simulink model "bb_core"  (R2025b)
settings: Solver=FixedStepDiscrete  StartTime=0.0  StopTime=0.035000000000000003  FixedStep=1/24e6  RelTol=1e-3
model workspace (MAT data in the model file):
  P_ABS_MAX_US = 2600
  P_ABS_MIN_US = 500
  P_CLK_PER_US = 24
  P_CMD = [165 11 0 10 164 165 141 0 0 40 165 0 3 231 64 165 143 0 0 42]
  P_CMD_T0 = 0.0005
  P_DEF_CENTER = 1750
  P_DEF_DSHIFT = 2
  P_DEF_ILIM = 200
  P_DEF_KD = 12800
  P_DEF_KI = 2
  P_DEF_KP = 768
  P_DEF_MANUAL = 1750
  P_DEF_MODE = 13
  P_DEF_SETPOINT = 330
  P_DEF_SMAX = 2500
  P_DEF_SMIN = 1000
  P_DEF_TRIG_MS = 40
  P_DT = 4.16666666667e-08
  P_ECHO_MAX_US = 30000
  P_INIT_US = 1750
  P_MAX_MM = 1000
  P_MIN_MM = 20
  P_MM_PER_US_Q16 = 11239
  P_PERIOD_US = 20000
  P_RISE_TMO_US = 10000
  P_TRIG_US = 12
  P_UART_DIV = 208
  P_VERSION = 47873
settings Model: Creator=Thanotos  LastModifiedBy=Thanotos
settings DebuggingCC: AlgebraicLoopMsg=error  SingleTaskRateTransMsg=error

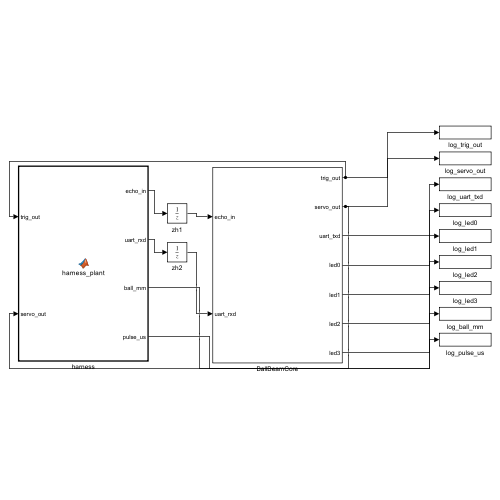
[thumbnail: Simulink's stored preview of the top-level diagram]
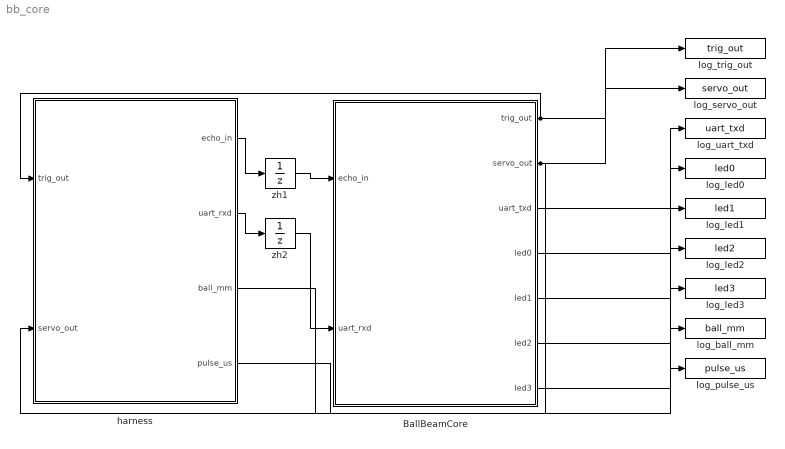
== system bb_core ==
  BallBeamCore : Subsystem
  harness : MATLAB Function  TreatAsAtomicUnit=on
  log_ball_mm : ToWorkspace  VariableName=ball_mm  SampleTime=-1
      settings: Decimation=2400
  log_led0 : ToWorkspace  VariableName=led0  SampleTime=-1
  log_led1 : ToWorkspace  VariableName=led1  SampleTime=-1
  log_led2 : ToWorkspace  VariableName=led2  SampleTime=-1
  log_led3 : ToWorkspace  VariableName=led3  SampleTime=-1
  log_pulse_us : ToWorkspace  VariableName=pulse_us  SampleTime=-1
      settings: Decimation=2400
  log_servo_out : ToWorkspace  VariableName=servo_out  SampleTime=-1
  log_trig_out : ToWorkspace  VariableName=trig_out  SampleTime=-1
  log_uart_txd : ToWorkspace  VariableName=uart_txd  SampleTime=-1
  zh1 : UnitDelay  SampleTime=-1  HasFrameUpgradeWarning=on
  zh2 : UnitDelay  InitialCondition=1  SampleTime=-1  HasFrameUpgradeWarning=on
  wires:
  harness/1(echo_in) -> zh1/1
  zh1/1 -> BallBeamCore/1(echo_in)
  harness/2(uart_rxd) -> zh2/1
  zh2/1 -> BallBeamCore/2(uart_rxd)
  BallBeamCore/1(trig_out) -> harness/1(trig_out), log_trig_out/1
  BallBeamCore/2(servo_out) -> harness/2(servo_out), log_servo_out/1
  BallBeamCore/3(uart_txd) -> log_uart_txd/1
  BallBeamCore/4(led0) -> log_led0/1
  BallBeamCore/5(led1) -> log_led1/1
  BallBeamCore/6(led2) -> log_led2/1
  BallBeamCore/7(led3) -> log_led3/1
  harness/3(ball_mm) -> log_ball_mm/1
  harness/4(pulse_us) -> log_pulse_us/1

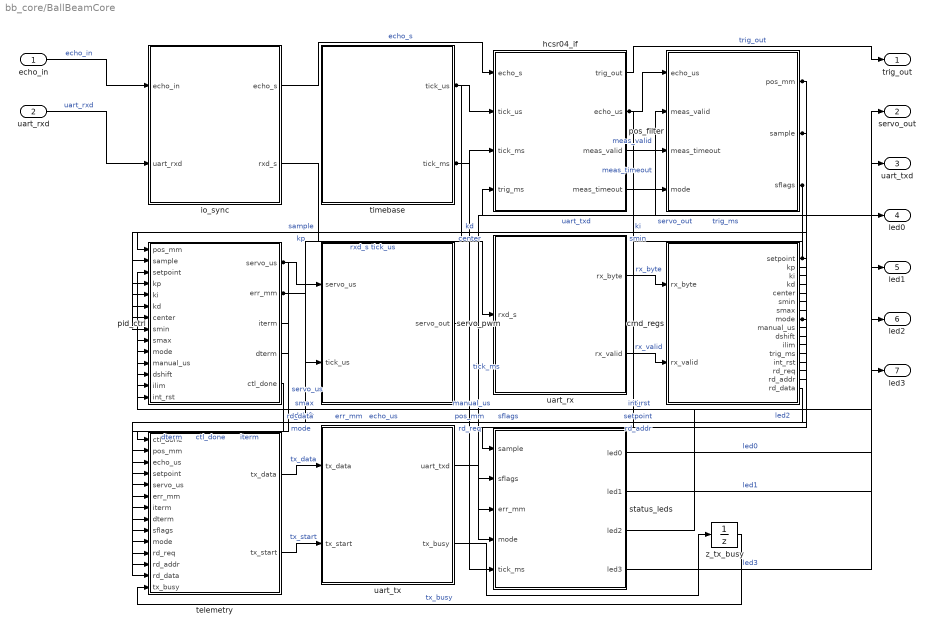
== system bb_core/BallBeamCore ==
  echo_in : Inport  OutDataTypeStr=boolean
  uart_rxd : Inport  Port=2  OutDataTypeStr=boolean
  cmd_regs : MATLAB Function  TreatAsAtomicUnit=on
  hcsr04_if : MATLAB Function  TreatAsAtomicUnit=on
  io_sync : MATLAB Function  TreatAsAtomicUnit=on
  pid_ctrl : MATLAB Function  TreatAsAtomicUnit=on
  pos_filter : MATLAB Function  TreatAsAtomicUnit=on
  servo_pwm : MATLAB Function  TreatAsAtomicUnit=on
  status_leds : MATLAB Function  TreatAsAtomicUnit=on
  telemetry : MATLAB Function  TreatAsAtomicUnit=on
  timebase : MATLAB Function  TreatAsAtomicUnit=on
  uart_rx : MATLAB Function  TreatAsAtomicUnit=on
  uart_tx : MATLAB Function  TreatAsAtomicUnit=on
  z_tx_busy : UnitDelay  SampleTime=-1  HasFrameUpgradeWarning=on
  trig_out : Outport
  servo_out : Outport  Port=2
  uart_txd : Outport  Port=3
  led0 : Outport  Port=4
  led1 : Outport  Port=5
  led2 : Outport  Port=6
  led3 : Outport  Port=7
  wires:
  echo_in/1 -> io_sync/1(echo_in)  "echo_in"
  uart_rxd/1 -> io_sync/2(uart_rxd)  "uart_rxd"
  io_sync/1(echo_s) -> hcsr04_if/1(echo_s)  "echo_s"
  timebase/1(tick_us) -> hcsr04_if/2(tick_us), servo_pwm/2(tick_us)  "tick_us"
  timebase/2(tick_ms) -> hcsr04_if/3(tick_ms), status_leds/5(tick_ms)  "tick_ms"
  cmd_regs/12(trig_ms) -> hcsr04_if/4(trig_ms)  "trig_ms"
  hcsr04_if/2(echo_us) -> pos_filter/1(echo_us), telemetry/3(echo_us)  "echo_us"
  hcsr04_if/3(meas_valid) -> pos_filter/2(meas_valid)  "meas_valid"
  hcsr04_if/4(meas_timeout) -> pos_filter/3(meas_timeout)  "meas_timeout"
  cmd_regs/8(mode) -> pos_filter/4(mode), pid_ctrl/10(mode), telemetry/10(mode), status_leds/4(mode)  "mode"
  pos_filter/1(pos_mm) -> pid_ctrl/1(pos_mm), telemetry/2(pos_mm)  "pos_mm"
  pos_filter/2(sample) -> pid_ctrl/2(sample), status_leds/1(sample)  "sample"
  cmd_regs/1(setpoint) -> pid_ctrl/3(setpoint), telemetry/4(setpoint)  "setpoint"
  cmd_regs/2(kp) -> pid_ctrl/4(kp)  "kp"
  cmd_regs/3(ki) -> pid_ctrl/5(ki)  "ki"
  cmd_regs/4(kd) -> pid_ctrl/6(kd)  "kd"
  cmd_regs/5(center) -> pid_ctrl/7(center)  "center"
  cmd_regs/6(smin) -> pid_ctrl/8(smin)  "smin"
  cmd_regs/7(smax) -> pid_ctrl/9(smax)  "smax"
  cmd_regs/9(manual_us) -> pid_ctrl/11(manual_us)  "manual_us"
  cmd_regs/10(dshift) -> pid_ctrl/12(dshift)  "dshift"
  cmd_regs/11(ilim) -> pid_ctrl/13(ilim)  "ilim"
  cmd_regs/13(int_rst) -> pid_ctrl/14(int_rst)  "int_rst"
  pid_ctrl/1(servo_us) -> servo_pwm/1(servo_us), telemetry/5(servo_us)  "servo_us"
  io_sync/2(rxd_s) -> uart_rx/1(rxd_s)  "rxd_s"
  uart_rx/1(rx_byte) -> cmd_regs/1(rx_byte)  "rx_byte"
  uart_rx/2(rx_valid) -> cmd_regs/2(rx_valid)  "rx_valid"
  pid_ctrl/5(ctl_done) -> telemetry/1(ctl_done)  "ctl_done"
  pid_ctrl/2(err_mm) -> telemetry/6(err_mm), status_leds/3(err_mm)  "err_mm"
  pid_ctrl/3(iterm) -> telemetry/7(iterm)  "iterm"
  pid_ctrl/4(dterm) -> telemetry/8(dterm)  "dterm"
  pos_filter/3(sflags) -> telemetry/9(sflags), status_leds/2(sflags)  "sflags"
  cmd_regs/14(rd_req) -> telemetry/11(rd_req)  "rd_req"
  cmd_regs/15(rd_addr) -> telemetry/12(rd_addr)  "rd_addr"
  cmd_regs/16(rd_data) -> telemetry/13(rd_data)  "rd_data"
  uart_tx/2(tx_busy) -> z_tx_busy/1
  z_tx_busy/1 -> telemetry/14(tx_busy)  "tx_busy"
  telemetry/1(tx_data) -> uart_tx/1(tx_data)  "tx_data"
  telemetry/2(tx_start) -> uart_tx/2(tx_start)  "tx_start"
  hcsr04_if/1(trig_out) -> trig_out/1  "trig_out"
  servo_pwm/1(servo_out) -> servo_out/1  "servo_out"
  uart_tx/1(uart_txd) -> uart_txd/1  "uart_txd"
  status_leds/1(led0) -> led0/1  "led0"
  status_leds/2(led1) -> led1/1  "led1"
  status_leds/3(led2) -> led2/1  "led2"
  status_leds/4(led3) -> led3/1  "led3"

== matlab function bb_core/BallBeamCore/servo_pwm ==
  settings: fimath=hdlfimath
  data: servo_us input uint16; servo_out output boolean; tick_us input boolean; P_PERIOD_US parameter; P_ABS_MIN_US parameter; P_ABS_MAX_US parameter; P_INIT_US parameter
function servo_out = servo_pwm(servo_us, tick_us, P_PERIOD_US, P_ABS_MIN_US, P_ABS_MAX_US, P_INIT_US)
%SERVO_PWM  50 Hz servo pulse with 1 us resolution. The width is latched
%   at the start of each period (glitch-free) and hard-clamped to a safe range.
%#codegen
persistent cnt width out
if isempty(cnt)
    cnt = uint16(0); width = uint16(P_INIT_US); out = false;
end
servo_out = out;
if tick_us
    if cnt >= uint16(P_PERIOD_US - 1)
        cnt = uint16(0);
        w = servo_us;
        if w < uint16(P_ABS_MIN_US), w = uint16(P_ABS_MIN_US); end
        if w > uint16(P_ABS_MAX_US), w = uint16(P_ABS_MAX_US); end
        width = w;
    else
        cnt = cnt + uint16(1);
    end
end
out = cnt < width;
end

== matlab function bb_core/BallBeamCore/uart_rx ==
  settings: fimath=hdlfimath
  data: rxd_s input boolean; rx_byte output uint8; rx_valid output boolean; P_UART_DIV parameter
function [rx_byte, rx_valid] = uart_rx(rxd_s, P_UART_DIV)
%UART_RX  8N1 receiver, samples each bit at its centre. rx_valid pulses
%   for one clock per good byte; bytes with a bad stop bit are dropped.
%#codegen
persistent st cnt bitn sh ob ov
if isempty(st)
    st = uint8(0); cnt = uint16(0); bitn = uint8(0); sh = uint8(0);
    ob = uint8(0); ov = false;
end
rx_byte  = ob;
rx_valid = ov;
ov = false;

if st == uint8(0)                       % idle, wait for start bit
    if ~rxd_s
        cnt = uint16(floor(P_UART_DIV/2));
        st = uint8(1);
    end
elseif st == uint8(1)                   % middle of start bit
    if cnt == uint16(0)
        if ~rxd_s
            cnt = uint16(P_UART_DIV - 1);
            bitn = uint8(0);
            st = uint8(2);
        else
            st = uint8(0);              % glitch
        end
    else
        cnt = cnt - uint16(1);
    end
elseif st == uint8(2)                   % data bits, LSB first
    if cnt == uint16(0)
        sh = bitshift(sh, -1);
        if rxd_s
            sh = bitor(sh, uint8(128));
        end
        cnt = uint16(P_UART_DIV - 1);
        if bitn == uint8(7)
            st = uint8(3);
        else
            bitn = bitn + uint8(1);
        end
    else
        cnt = cnt - uint16(1);
    end
elseif st == uint8(3)                   % stop bit
    if cnt == uint16(0)
        if rxd_s
            ob = sh;
            ov = true;
            st = uint8(0);
        else
            st = uint8(4);              % framing error
        end
    else
        cnt = cnt - uint16(1);
    end
else                                    % 4: wait for line idle
    if rxd_s
        st = uint8(0);
    end
end
end

== matlab function bb_core/BallBeamCore/cmd_regs ==
  settings: fimath=hdlfimath
  data: rx_byte input uint8; setpoint output uint16; rx_valid input boolean; kp output uint16; ki output uint16; kd output uint16; center output uint16; smin output uint16; smax output uint16; mode output uint16; manual_us output uint16; dshift output uint16; ilim output uint16; trig_ms output uint16; int_rst output boolean; rd_req output boolean; rd_addr output uint8; rd_data output uint16; P_DEF_SETPOINT parameter; P_DEF_KP parameter; P_DEF_KI parameter; P_DEF_KD parameter; P_DEF_CENTER parameter; P_DEF_SMIN parameter; P_DEF_SMAX parameter; P_DEF_MODE parameter; P_DEF_MANUAL parameter; P_DEF_DSHIFT parameter; P_DEF_ILIM parameter; P_DEF_TRIG_MS parameter; P_VERSION parameter
function [setpoint, kp, ki, kd, center, smin, smax, mode, manual_us, dshift, ilim, trig_ms, ...
    int_rst, rd_req, rd_addr, rd_data] = cmd_regs(rx_byte, rx_valid, ...
    P_DEF_SETPOINT, P_DEF_KP, P_DEF_KI, P_DEF_KD, P_DEF_CENTER, P_DEF_SMIN, P_DEF_SMAX, ...
P_DEF_MODE, P_DEF_MANUAL, P_DEF_DSHIFT, P_DEF_ILIM, P_DEF_TRIG_MS, P_VERSION)
%CMD_REGS  UART command parser + register file.
%   Host frame (5 bytes):  A5  ADDR  HI  LO  CHK,   CHK = A5^ADDR^HI^LO
%     ADDR bit7 = 0 : write HI:LO to register ADDR
%     ADDR bit7 = 1 : read register ADDR&7F (HI/LO ignored) -> reply frame
%   Registers: 00 setpoint mm | 01 Kp | 02 Ki | 03 Kd (Q8.8)
%     04 servo centre us | 05 servo min | 06 servo max | 07 mode
%     08 manual servo us | 09 D filter shift | 0A integrator limit us
%     0B trigger period ms | 0C write: bit0 = reset integrator
%     0D version (RO) | 0E good frames (RO) | 0F bad-checksum frames (RO)
%   A partial frame is discarded after 65535 clocks (~2.7 ms) of silence.
%#codegen
persistent st a hi lo tmo r_sp r_kp r_ki r_kd r_c r_mn r_mx r_md r_man r_ds r_il r_tr ...
    n_ok n_bad irst rq ra rdat
if isempty(st)
    st = uint8(0); a = uint8(0); hi = uint8(0); lo = uint8(0); tmo = uint16(0);
    r_sp = uint16(P_DEF_SETPOINT); r_kp = uint16(P_DEF_KP); r_ki = uint16(P_DEF_KI);
    r_kd = uint16(P_DEF_KD); r_c = uint16(P_DEF_CENTER); r_mn = uint16(P_DEF_SMIN);
    r_mx = uint16(P_DEF_SMAX); r_md = uint16(P_DEF_MODE); r_man = uint16(P_DEF_MANUAL);
    r_ds = uint16(P_DEF_DSHIFT); r_il = uint16(P_DEF_ILIM); r_tr = uint16(P_DEF_TRIG_MS);
    n_ok = uint16(0); n_bad = uint16(0); irst = false; rq = false; ra = uint8(0); rdat = uint16(0);
end
setpoint = r_sp; kp = r_kp; ki = r_ki; kd = r_kd; center = r_c; smin = r_mn; smax = r_mx;
mode = r_md; manual_us = r_man; dshift = r_ds; ilim = r_il; trig_ms = r_tr;
int_rst = irst; rd_req = rq; rd_addr = ra; rd_data = rdat;

irst = false;
rq = false;

if rx_valid
    tmo = uint16(0);
    if st == uint8(0)
        if rx_byte == uint8(165)        % 0xA5
            st = uint8(1);
        end
    elseif st == uint8(1)
        a = rx_byte; st = uint8(2);
    elseif st == uint8(2)
        hi = rx_byte; st = uint8(3);
    elseif st == uint8(3)
        lo = rx_byte; st = uint8(4);
    else
        st = uint8(0);
        chk = bitxor(bitxor(uint8(165), a), bitxor(hi, lo));
        if chk == rx_byte
            if n_ok < uint16(65535), n_ok = n_ok + uint16(1); end
            v = bitor(bitshift(uint16(hi), 8), uint16(lo));
            if bitand(a, uint8(128)) ~= uint8(0)
                ra = bitand(a, uint8(127));
                rq = true;
            else
                if a == uint8(0),  r_sp = v; end
                if a == uint8(1),  r_kp = v; end
                if a == uint8(2),  r_ki = v; end
                if a == uint8(3),  r_kd = v; end
                if a == uint8(4),  r_c  = v; end
                if a == uint8(5),  r_mn = v; end
                if a == uint8(6),  r_mx = v; end
                if a == uint8(7),  r_md = v; end
                if a == uint8(8),  r_man = v; end
                if a == uint8(9),  r_ds = bitand(v, uint16(7)); end
                if a == uint8(10), r_il = v; end
                if a == uint8(11), r_tr = v; end
                if a == uint8(12), irst = bitand(v, uint16(1)) ~= uint16(0); end
            end
        else
            if n_bad < uint16(65535), n_bad = n_bad + uint16(1); end
        end
    end
else
    if st ~= uint8(0)
        if tmo == uint16(65535)
            st = uint8(0);
            tmo = uint16(0);
        else
            tmo = tmo + uint16(1);
        end
    end
end

% read mux (registered; valid together with rd_req)
ad = bitand(a, uint8(127));
if ad == uint8(0),      rdat = r_sp;
elseif ad == uint8(1),  rdat = r_kp;
elseif ad == uint8(2),  rdat = r_ki;
elseif ad == uint8(3),  rdat = r_kd;
elseif ad == uint8(4),  rdat = r_c;
elseif ad == uint8(5),  rdat = r_mn;
elseif ad == uint8(6),  rdat = r_mx;
elseif ad == uint8(7),  rdat = r_md;
elseif ad == uint8(8),  rdat = r_man;
elseif ad == uint8(9),  rdat = r_ds;
elseif ad == uint8(10), rdat = r_il;
elseif ad == uint8(11), rdat = r_tr;
elseif ad == uint8(13), rdat = uint16(P_VERSION);
elseif ad == uint8(14), rdat = n_ok;
elseif ad == uint8(15), rdat = n_bad;
else,                   rdat = uint16(0);
end
end

== matlab function bb_core/BallBeamCore/telemetry ==
  settings: fimath=hdlfimath
  data: ctl_done input boolean; tx_data output uint8; pos_mm input uint16; echo_us input uint16; setpoint input uint16; servo_us input uint16; err_mm input int16; iterm input int16; dterm input int16; sflags input uint8; mode input uint16; rd_req input boolean; rd_addr input uint8; rd_data input uint16; tx_busy input boolean; tx_start output boolean
function [tx_data, tx_start] = telemetry(ctl_done, pos_mm, echo_us, setpoint, servo_us, err_mm, iterm, dterm, ...
    sflags, mode, rd_req, rd_addr, rd_data, tx_busy)
%TELEMETRY  Serialises frames to the UART transmitter.
%   Telemetry (19 bytes, after every control update when mode bit2 = 1):
%     5A 10 SEQ POS(2) ECHO_US(2) SETPOINT(2) SERVO_US(2) ERR(2) I(2) D(2) FLAGS CHK
%   Register read reply (6 bytes):  5A 20 ADDR HI LO CHK
%   Multi-byte fields are big-endian; ERR/I/D are int16. CHK = XOR of all
%   previous bytes of the frame. FLAGS: bit0 echo timeout, bit1 out of
%   range, bit2 loop enabled, bit3 inverted, bit4 median filter on.
%#codegen
persistent st idx len wt seq b data_r start_r prd pa pd
if isempty(st)
    st = uint8(0); idx = uint8(0); len = uint8(0); wt = uint8(0); seq = uint8(0);
    b = zeros(1, 19, 'uint8'); data_r = uint8(0); start_r = false;
    prd = false; pa = uint8(0); pd = uint16(0);
end
tx_data  = data_r;
tx_start = start_r;
start_r  = false;

if rd_req
    prd = true; pa = rd_addr; pd = rd_data;
end

if st == uint8(0)
    if ctl_done && bitand(mode, uint16(4)) ~= uint16(0)
        fl = bitand(sflags, uint8(3));
        if bitand(mode, uint16(1)) ~= uint16(0), fl = bitor(fl, uint8(4)); end
        if bitand(mode, uint16(2)) ~= uint16(0), fl = bitor(fl, uint8(8)); end
        if bitand(mode, uint16(8)) ~= uint16(0), fl = bitor(fl, uint8(16)); end
        e16 = s2u(err_mm); i16 = s2u(iterm); d16 = s2u(dterm);
        b(1) = uint8(90);  b(2) = uint8(16); b(3) = seq;
        b(4) = hb(pos_mm);   b(5) = lb(pos_mm);
        b(6) = hb(echo_us);  b(7) = lb(echo_us);
        b(8) = hb(setpoint); b(9) = lb(setpoint);
        b(10) = hb(servo_us); b(11) = lb(servo_us);
        b(12) = hb(e16); b(13) = lb(e16);
        b(14) = hb(i16); b(15) = lb(i16);
        b(16) = hb(d16); b(17) = lb(d16);
        b(18) = fl;
        c = uint8(0);
        for k = 1:18
            c = bitxor(c, b(k));
        end
        b(19) = c;
        seq = seq + uint8(1);
        len = uint8(19); idx = uint8(0); st = uint8(1);
    elseif prd
        prd = false;
        b(1) = uint8(90); b(2) = uint8(32); b(3) = pa; b(4) = hb(pd); b(5) = lb(pd);
        b(6) = bitxor(bitxor(bitxor(b(1), b(2)), bitxor(b(3), b(4))), b(5));
        len = uint8(6); idx = uint8(0); st = uint8(1);
    end
elseif st == uint8(1)                   % hand next byte to the UART
    if ~tx_busy
        data_r  = b(idx + 1);
        start_r = true;
        wt = uint8(3);
        st = uint8(2);
    end
else                                    % 2: let tx_busy assert
    if wt == uint8(0)
        idx = idx + uint8(1);
        if idx == len
            st = uint8(0);
        else
            st = uint8(1);
        end
    else
        wt = wt - uint8(1);
    end
end
end

function y = hb(x)
y = uint8(bitshift(x, -8));
end

function y = lb(x)
y = uint8(bitand(x, uint16(255)));
end

function y = s2u(x)
% int16 -> uint16 two's-complement bit pattern
if x < int16(0)
    y = uint16(int32(x) + int32(65536));
else
    y = uint16(x);
end
end

== matlab function bb_core/BallBeamCore/uart_tx ==
  settings: fimath=hdlfimath
  data: tx_data input uint8; uart_txd output boolean; tx_start input boolean; tx_busy output boolean; P_UART_DIV parameter
function [uart_txd, tx_busy] = uart_tx(tx_data, tx_start, P_UART_DIV)
%UART_TX  8N1 transmitter. tx_start is accepted only while idle.
%#codegen
persistent st cnt bitn sh line busy
if isempty(st)
    st = uint8(0); cnt = uint16(0); bitn = uint8(0); sh = uint8(0);
    line = true; busy = false;
end
uart_txd = line;
tx_busy  = busy;

if st == uint8(0)
    line = true;
    if tx_start
        sh   = tx_data;
        line = false;                   % start bit
        cnt  = uint16(P_UART_DIV - 1);
        st   = uint8(1);
        busy = true;
    else
        busy = false;
    end
elseif st == uint8(1)                   % end of start bit -> bit 0
    if cnt == uint16(0)
        line = bitand(sh, uint8(1)) ~= uint8(0);
        sh   = bitshift(sh, -1);
        bitn = uint8(0);
        cnt  = uint16(P_UART_DIV - 1);
        st   = uint8(2);
    else
        cnt = cnt - uint16(1);
    end
elseif st == uint8(2)                   % data bits 1..7, then stop
    if cnt == uint16(0)
        if bitn == uint8(6)
            line = bitand(sh, uint8(1)) ~= uint8(0);
            bitn = uint8(7);
        elseif bitn == uint8(7)
            line = true;                % stop bit
            st   = uint8(3);
        else
            line = bitand(sh, uint8(1)) ~= uint8(0);
            bitn = bitn + uint8(1);
        end
        sh  = bitshift(sh, -1);
        cnt = uint16(P_UART_DIV - 1);
    else
        cnt = cnt - uint16(1);
    end
else                                    % 3: stop bit
    if cnt == uint16(0)
        st = uint8(0);
    else
        cnt = cnt - uint16(1);
    end
end
end

== matlab function bb_core/BallBeamCore/status_leds ==
  settings: fimath=hdlfimath
  data: sample input boolean; led0 output boolean; sflags input uint8; err_mm input int16; mode input uint16; tick_ms input boolean; led1 output boolean; led2 output boolean; led3 output boolean
function [led0, led1, led2, led3] = status_leds(sample, sflags, err_mm, mode, tick_ms)
%STATUS_LEDS  led0: 30 ms flash per sensor sample   led1: |error| <= 10 mm
%             led2: last reading bad (timeout / out of range)
%             led3: 1 Hz heartbeat (fast 4 Hz blink when loop disabled)
%#codegen
persistent fl_cnt hb_cnt hb l0 l1 l2
if isempty(fl_cnt)
    fl_cnt = uint8(0); hb_cnt = uint16(0); hb = false; l0 = false; l1 = false; l2 = false;
end
led0 = l0; led1 = l1; led2 = l2; led3 = hb;

if sample
    fl_cnt = uint8(30);
    l2 = sflags ~= uint8(0);
elseif tick_ms && fl_cnt ~= uint8(0)
    fl_cnt = fl_cnt - uint8(1);
end
l0 = fl_cnt ~= uint8(0);
l1 = (err_mm <= int16(10)) && (err_mm >= int16(-10)) && ~l2;
if bitand(mode, uint16(1)) ~= uint16(0)
    half = uint16(499);
else
    half = uint16(124);
end
if tick_ms
    if hb_cnt >= half
        hb_cnt = uint16(0);
        hb = ~hb;
    else
        hb_cnt = hb_cnt + uint16(1);
    end
end
end

== matlab function bb_core/harness ==
  settings: fimath=hdlfimath
  data: trig_out input boolean; echo_in output boolean; servo_out input boolean; uart_rxd output boolean; ball_mm output double; pulse_us output double; P_DT parameter; P_CMD parameter; P_CMD_T0 parameter; P_UART_DIV parameter
function [echo_in, uart_rxd, ball_mm, pulse_us] = harness_plant(trig_out, servo_out, P_DT, P_CMD, P_CMD_T0, P_UART_DIV)
%HARNESS_PLANT  Test-bench only (not converted to HDL).
%   * HC-SR04 model: 200 us after the trigger falls, echo goes high for
%     2*x/343 m/s.
%   * Ball-and-beam plant (bb_plant_step equations) driven by the measured
%     servo pulse width.
%   * UART host: sends the byte list P_CMD at 115200 8N1 starting at P_CMD_T0.
%#codegen
persistent t trig_d echo_t0 echo_t1 x v th hi_t pw bi bitpos bitcnt line
if isempty(t)
    t = 0; trig_d = false; echo_t0 = -1; echo_t1 = -1;
    x = 0.15; v = 0; th = 0; hi_t = 0; pw = 1750;
    bi = 1; bitpos = -1; bitcnt = 0; line = true;
end
pl.center_us = 1750; pl.rad_per_us = 0.1*0.09*pi/180; pl.tau_servo = 0.03;
pl.slew_us_per_s = 6000; pl.xmin = 0.04; pl.xmax = 0.60;

% outputs from current state
echo_in  = (t >= echo_t0) && (t < echo_t1);
uart_rxd = line;
ball_mm  = x*1000;
pulse_us = pw;

% ---- sensor ----
if trig_d && ~trig_out
    echo_t0 = t + 200e-6;
    echo_t1 = echo_t0 + 2*x/343;
end
trig_d = trig_out;

% ---- servo pulse measurement ----
if servo_out
    hi_t = hi_t + P_DT;
elseif hi_t > 0
    pw = hi_t*1e6; hi_t = 0;
end

% ---- plant (bb_plant_step inlined) ----
target = pw - pl.center_us;
dth = (target - th)/pl.tau_servo*P_DT;
maxd = pl.slew_us_per_s*P_DT;
dth = max(-maxd, min(maxd, dth));
th = th + dth;
a = (5/7)*9.81*sin(pl.rad_per_us*th);
v = v + a*P_DT; x = x + v*P_DT;
if x < pl.xmin, x = pl.xmin; v = 0; end
if x > pl.xmax, x = pl.xmax; v = 0; end

% ---- UART host transmitter (clock-count based, like the RTL) ----
if t >= P_CMD_T0 && bi <= numel(P_CMD)
    if bitpos < 0
        bitpos = 0; bitcnt = 0;
    end
    if bitcnt == 0
        if bitpos == 0
            line = false;                               % start
        elseif bitpos <= 8
            line = bitand(bitshift(P_CMD(bi), -(bitpos-1)), 1) ~= 0;
        else
            line = true;                                % stop + 1 bit gap
        end
    end
    bitcnt = bitcnt + 1;
    if bitcnt >= P_UART_DIV
        bitcnt = 0; bitpos = bitpos + 1;
        if bitpos > 10
            bitpos = -1; bi = bi + 1;
        end
    end
end
t = t + P_DT;
end

== matlab function bb_core/BallBeamCore/timebase ==
  settings: fimath=hdlfimath
  data: tick_us output boolean; tick_ms output boolean; P_CLK_PER_US parameter
function [tick_us, tick_ms] = timebase(P_CLK_PER_US)
%TIMEBASE  1 us and 1 ms clock-enable strobes (one clock wide).
%#codegen
persistent c_clk c_us t_us t_ms
if isempty(c_clk)
    c_clk = uint8(0); c_us = uint16(0); t_us = false; t_ms = false;
end
tick_us = t_us;
tick_ms = t_ms;
if c_clk == uint8(P_CLK_PER_US - 1)
    c_clk = uint8(0);
    t_us  = true;
    if c_us == uint16(999)
        c_us = uint16(0);
        t_ms = true;
    else
        c_us = c_us + uint16(1);
        t_ms = false;
    end
else
    c_clk = c_clk + uint8(1);
    t_us  = false;
    t_ms  = false;
end
end

== matlab function bb_core/BallBeamCore/io_sync ==
  settings: fimath=hdlfimath
  data: echo_in input boolean; echo_s output boolean; uart_rxd input boolean; rxd_s output boolean
function [echo_s, rxd_s] = io_sync(echo_in, uart_rxd)
%IO_SYNC  Two-flop synchronisers for the asynchronous inputs.
%#codegen
persistent e1 e2 r1 r2
if isempty(e1)
    e1 = false; e2 = false; r1 = true; r2 = true;
end
echo_s = e2;
rxd_s  = r2;
e2 = e1; e1 = echo_in;
r2 = r1; r1 = uart_rxd;
end

== matlab function bb_core/BallBeamCore/hcsr04_if ==
  settings: fimath=hdlfimath
  data: echo_s input boolean; trig_out output boolean; tick_us input boolean; tick_ms input boolean; trig_ms input uint16; echo_us output uint16; meas_valid output boolean; meas_timeout output boolean; P_TRIG_US parameter; P_RISE_TMO_US parameter; P_ECHO_MAX_US parameter
function [trig_out, echo_us, meas_valid, meas_timeout] = hcsr04_if(echo_s, tick_us, tick_ms, trig_ms, ...
    P_TRIG_US, P_RISE_TMO_US, P_ECHO_MAX_US)
%HCSR04_IF  Triggers the HC-SR04 every trig_ms (>=10 ms, and never before the
%   previous echo has finished) and measures the echo high time in us.
%   meas_valid pulses once per measurement attempt; meas_timeout marks a
%   missing / too-long echo (echo_us is then not a distance).
%#codegen
persistent st ms_cnt us_cnt echo_d trig_r out_us out_v out_to
if isempty(st)
    st = uint8(0); ms_cnt = uint16(0); us_cnt = uint16(0); echo_d = false;
    trig_r = false; out_us = uint16(0); out_v = false; out_to = false;
end
trig_out     = trig_r;
echo_us      = out_us;
meas_valid   = out_v;
meas_timeout = out_to;

out_v = false;
period = trig_ms;
if period < uint16(10)
    period = uint16(10);
end
if tick_ms && ms_cnt < uint16(1000)
    ms_cnt = ms_cnt + uint16(1);
end
rise = echo_s && ~echo_d;
fall = ~echo_s && echo_d;
echo_d = echo_s;

if st == uint8(0)                       % IDLE: wait for the period
    if ms_cnt >= period
        ms_cnt = uint16(0);
        us_cnt = uint16(0);
        trig_r = true;
        st = uint8(1);
    end
elseif st == uint8(1)                   % TRIG: hold trigger high
    if tick_us
        if us_cnt >= uint16(P_TRIG_US - 1)
            trig_r = false;
            us_cnt = uint16(0);
            st = uint8(2);
        else
            us_cnt = us_cnt + uint16(1);
        end
    end
elseif st == uint8(2)                   % WAIT for echo rising edge
    if rise
        us_cnt = uint16(0);
        st = uint8(3);
    elseif tick_us
        if us_cnt >= uint16(P_RISE_TMO_US)
            out_us = uint16(0);
            out_to = true;
            out_v  = true;
            st = uint8(0);
        else
            us_cnt = us_cnt + uint16(1);
        end
    end
elseif st == uint8(3)                   % MEASURE echo high time
    if fall
        out_us = us_cnt;
        out_to = false;
        out_v  = true;
        st = uint8(0);
    elseif tick_us
        if us_cnt >= uint16(P_ECHO_MAX_US)
            out_us = us_cnt;
            out_to = true;
            out_v  = true;
            st = uint8(4);
        else
            us_cnt = us_cnt + uint16(1);
        end
    end
else                                    % 4: echo stuck high, wait for low
    if ~echo_s
        st = uint8(0);
    end
end
end

== matlab function bb_core/BallBeamCore/pos_filter ==
  settings: fimath=hdlfimath
  data: echo_us input uint16; pos_mm output uint16; meas_valid input boolean; meas_timeout input boolean; mode input uint16; sample output boolean; sflags output uint8; P_MM_PER_US_Q16 parameter; P_MIN_MM parameter; P_MAX_MM parameter
function [pos_mm, sample, sflags] = pos_filter(echo_us, meas_valid, meas_timeout, mode, ...
    P_MM_PER_US_Q16, P_MIN_MM, P_MAX_MM)
%POS_FILTER  Echo time -> millimetres, range check, optional median-of-3.
%   Emits one `sample` strobe per measurement attempt so the controller
%   runs at a fixed rate. Bad readings hold the last good position.
%   sflags: bit0 = echo timeout, bit1 = out of range.
%#codegen
persistent h0 h1 h2 last have out_pos out_s out_f
if isempty(h0)
    h0 = uint16(0); h1 = uint16(0); h2 = uint16(0); last = uint16(0);
    have = false; out_pos = uint16(0); out_s = false; out_f = uint8(0);
end
pos_mm = out_pos;
sample = out_s;
sflags = out_f;

out_s = false;
if meas_valid
    prod = uint32(echo_us) * uint32(P_MM_PER_US_Q16);
    mm   = uint16(bitshift(prod, -16));
    inrange = (mm >= uint16(P_MIN_MM)) && (mm <= uint16(P_MAX_MM));
    if meas_timeout
        out_f = uint8(1);
    elseif ~inrange
        out_f = uint8(2);
    else
        out_f = uint8(0);
        if have
            h2 = h1; h1 = h0; h0 = mm;
        else
            h2 = mm; h1 = mm; h0 = mm; have = true;
        end
        if bitand(mode, uint16(8)) ~= uint16(0)
            mn = min(h0, h1);
            mx = max(h0, h1);
            last = max(mn, min(mx, h2));
        else
            last = mm;
        end
    end
    out_pos = last;
    out_s = true;
end
end

== matlab function bb_core/BallBeamCore/pid_ctrl ==
  settings: fimath=hdlfimath
  data: pos_mm input uint16; servo_us output uint16; sample input boolean; setpoint input uint16; kp input uint16; ki input uint16; kd input uint16; center input uint16; smin input uint16; smax input uint16; mode input uint16; manual_us input uint16; dshift input uint16; ilim input uint16; int_rst input boolean; err_mm output int16; iterm output int16; dterm output int16; ctl_done output boolean
function [servo_us, err_mm, iterm, dterm, ctl_done] = pid_ctrl(pos_mm, sample, setpoint, kp, ki, kd, ...
    center, smin, smax, mode, manual_us, dshift, ilim, int_rst)
%PID_CTRL  Discrete PID, executed once per sensor sample (4-cycle sequence,
%   one shared multiplier).
%     e  = setpoint - pos                     [mm]
%     P  = Kp*e
%     I += Ki*e,  clamped to +/- ilim us      (anti-windup)
%     D  = Kd*filt(pos[k-1]-pos[k])           (derivative on measurement,
%                                              IIR alpha = 1/2^dshift)
%     servo = clamp(center +/- (P+I+D), smin, smax)
%   Gains are Q8.8; internal sums are in us*256.
%   mode bit0 = loop enable (else servo = manual_us), bit1 = invert output.
%   Bit-exact sample-level reference: bb_ctrl_ref.m.
%#codegen
persistent stg have pos_prev df e_r iacc pacc dacc servo_r err_r it_r dt_r done_r
if isempty(stg)
    stg = uint8(0); have = false; pos_prev = uint16(0); df = int32(0); e_r = int32(0);
    iacc = int32(0); pacc = int32(0); dacc = int32(0);
    servo_r = uint16(1750); err_r = int16(0); it_r = int16(0); dt_r = int16(0); done_r = false;
end
servo_us = servo_r;
err_mm   = err_r;
iterm    = it_r;
dterm    = dt_r;
ctl_done = done_r;

done_r = false;
enable = bitand(mode, uint16(1)) ~= uint16(0);
invert = bitand(mode, uint16(2)) ~= uint16(0);

% ---- shared multiplier: operand select by stage ----
if stg == uint8(1)
    ma = int32(kp);  mb = e_r;
elseif stg == uint8(2)
    ma = int32(ki);  mb = e_r;
else
    ma = int32(kd);  mb = df;
end
prod = ma * mb;

if stg == uint8(0)
    if sample
        e = int32(setpoint) - int32(pos_mm);
        if e > int32(2000), e = int32(2000); end
        if e < int32(-2000), e = int32(-2000); end
        if have
            dm = int32(pos_prev) - int32(pos_mm);
        else
            dm = int32(0);
        end
        if dm > int32(127), dm = int32(127); end
        if dm < int32(-127), dm = int32(-127); end
        have = true;
        pos_prev = pos_mm;
        x = dm*int32(256) - df;
        if dshift == uint16(0)
            df = df + x;
        elseif dshift == uint16(1)
            df = df + bitsra(x, 1);
        elseif dshift == uint16(2)
            df = df + bitsra(x, 2);
        elseif dshift == uint16(3)
            df = df + bitsra(x, 3);
        elseif dshift == uint16(4)
            df = df + bitsra(x, 4);
        elseif dshift == uint16(5)
            df = df + bitsra(x, 5);
        elseif dshift == uint16(6)
            df = df + bitsra(x, 6);
        else
            df = df + bitsra(x, 7);
        end
        e_r = e;
        stg = uint8(1);
    end
elseif stg == uint8(1)                  % P = Kp*e
    pacc = prod;
    stg = uint8(2);
elseif stg == uint8(2)                  % I += Ki*e
    lim = int32(ilim) * int32(256);
    inew = iacc + prod;
    if inew > lim, inew = lim; end
    if inew < -lim, inew = -lim; end
    if enable
        iacc = inew;
    else
        iacc = int32(0);
    end
    stg = uint8(3);
else                                    % 3: D = Kd*df, combine, clamp
    dacc = bitsra(prod, 8);
    u = bitsra(pacc + iacc + dacc, 8);
    if u > int32(4000), u = int32(4000); end
    if u < int32(-4000), u = int32(-4000); end
    if invert, u = -u; end
    if enable
        out = int32(center) + u;
    else
        out = int32(manual_us);
    end
    if out > int32(smax), out = int32(smax); end
    if out < int32(smin), out = int32(smin); end
    servo_r = uint16(out);
    err_r = int16(e_r);
    it_r  = int16(bitsra(iacc, 8));
    dv = bitsra(dacc, 8);
    if dv > int32(32767), dv = int32(32767); end
    if dv < int32(-32768), dv = int32(-32768); end
    dt_r = int16(dv);
    done_r = true;
    stg = uint8(0);
end
if int_rst
    iacc = int32(0);
end
end
